simulink model "GFMUPS100k_CPP"  (R2024b)
settings: Solver=ode2  StartTime=0.0  StopTime=6  FixedStep=5e-7  RelTol=1e-3
model workspace (MAT data in the model file):
  amp = 0
  f1 = 1000
undefined symbols (not defined in the file or in its folder): DiscIntNeverNeededParam, L
libraries: spsIGBTDiodeLib x12, slpidlib x12, spsabctodq0Lib x10, spsSeriesRLCBranchLib x9, spsPLL3phLib x8, spsThreePhaseSeriesRLCBranchLib x8, spsDiodeLib x6, dspstat3 x5, spsVoltageMeasurementLib x4, spsThreePhaseVIMeasurementLib x4, spsPower3phInstantaneousLib x3, spsControlledCurrentSourceLib x3
(part 4 of 4)

== matlab function GFMUPS100k_CPP/A practical and fast sequence components detection scheme for three-phase unbalanced grid voltage.2021/Ubeta计算/MATLAB Function9 ==
  data: u_alpha input; u_beta output; Ts input; omega input; N input
function u_beta = MultiPoint_OSG(u_alpha, Ts, omega, N)
% MULTIPOINT_OSG: 基于多点最小二乘最优拟合的正交信号构造
% 
% 参数说明:
%   u_alpha : 当前时刻的单相采样输入 u(k)
%   Ts      : 采样周期 (例如 1e-4)
%   omega   : 电网基波角频率 (例如 2*pi*50)
%   N       : 拟合使用的总点数 (建议值：4 代表4点拟合；21 代表2毫秒全密集拟合)

% 声明持久变量：历史缓冲区、常数系数数组、初始化标志
persistent u_buffer C_coeffs initialized;

% 初始化模块 (仅在系统启动的第一个采样周期执行一次，极大节省算力)
if isempty(initialized)
    % 1. 计算相邻采样点的电角度步长
    alpha = omega * Ts;
    
    % 2. 预生成约束矩阵的三角函数项
    c = zeros(N, 1);
    s = zeros(N, 1);
    for i = 1:N
        c(i) = cos((i-1) * alpha);
        s(i) = sin((i-1) * alpha);
    end
    
    % 3. 计算中间常数矩阵
    M11 = sum(c.^2);
    M12 = sum(c .* s);
    M22 = sum(s.^2);
    Delta = M11 * M22 - M12^2;
    
    % 4. 计算最优抗噪系数 C0, C1 ... C_N-1
    C_coeffs = zeros(N, 1);
    for i = 1:N
        C_coeffs(i) = (M12 * c(i) - M11 * s(i)) / Delta;
    end
    
    % 【极性匹配说明】
    % 您原先的代码 u_beta = (u(k-1) - u(k)*cos)/sin 
    % 在输入为 sin(wt) 时，输出的是 -cos(wt)。
    % 为了确保替换后系统后续的 PLL 或控制逻辑不受极性翻转的影响，这里乘以 -1。
    C_coeffs = -C_coeffs; 
    
    % 5. 初始化历史数据移位寄存器 (全 0)
    u_buffer = zeros(N, 1);
    initialized = true;
end

% ================= 实 时 运 行 区 =================

% 1. 更新历史数据缓冲区 (FIFO 移位)
% 将旧数据向后平移，新数据 u_alpha 推入头部 (u_buffer(1) 代表当前 k 时刻)
for i = N:-1:2
    u_buffer(i) = u_buffer(i-1);
end
u_buffer(1) = u_alpha;

% 2. 核心正交计算 (向量内积乘加运算)
% 等效于: u_beta = C0*u(k) + C1*u(k-1) + C2*u(k-2) + ...
u_beta = sum(C_coeffs .* u_buffer);

end

== matlab function GFMUPS100k_CPP/A practical and fast sequence components detection scheme for three-phase unbalanced grid voltage.2021/Subsystem/MATLAB Function1 ==
  settings: updateMethod=DISCRETE
  data: u input; y_out output
function y_out = maf_filter(u)
    % 滑动平均滤波法 (MAF)
    % 采样时间: 1e-4 s, 电网基波频率: 50 Hz
    % 窗口长度 L: T/2 = 0.01 s -> 100 个采样点 (用于消除 3, 5, 7 次等奇次谐波)
    
    % 定义持久化变量
    persistent buf_maf sum_maf idx_maf
    
    if isempty(buf_maf)
        buf_maf = zeros(100, 1);
        sum_maf = 0;
        idx_maf = 1;
    end
    
    % 读取窗口中最旧的值，即公式 (41) 中的 u(t - L*DeltaT)
    u_old = buf_maf(idx_maf);
    
    % 采用递推方式更新滑动窗口的总和，大幅降低每步运算量
    sum_maf = sum_maf + u - u_old; 
    
    % 计算当前步的平均值
    y_out = sum_maf / 100;
    
    % 更新环形缓冲区
    buf_maf(idx_maf) = u;
    
    % 更新索引
    idx_maf = idx_maf + 1;
    if idx_maf > 100
        idx_maf = 1;
    end
end

== matlab function GFMUPS100k_CPP/A practical and fast sequence components detection scheme for three-phase unbalanced grid voltage.2021/Subsystem/MATLAB Function2 ==
  settings: updateMethod=DISCRETE
  data: u input; y_out output
function y_out = maf_filter(u)
    % 滑动平均滤波法 (MAF)
    % 采样时间: 1e-4 s, 电网基波频率: 50 Hz
    % 窗口长度 L: T/2 = 0.01 s -> 100 个采样点 (用于消除 3, 5, 7 次等奇次谐波)
    
    % 定义持久化变量
    persistent buf_maf sum_maf idx_maf
    
    if isempty(buf_maf)
        buf_maf = zeros(100, 1);
        sum_maf = 0;
        idx_maf = 1;
    end
    
    % 读取窗口中最旧的值，即公式 (41) 中的 u(t - L*DeltaT)
    u_old = buf_maf(idx_maf);
    
    % 采用递推方式更新滑动窗口的总和，大幅降低每步运算量
    sum_maf = sum_maf + u - u_old; 
    
    % 计算当前步的平均值
    y_out = sum_maf / 100;
    
    % 更新环形缓冲区
    buf_maf(idx_maf) = u;
    
    % 更新索引
    idx_maf = idx_maf + 1;
    if idx_maf > 100
        idx_maf = 1;
    end
end

== matlab function GFMUPS100k_CPP/A practical and fast sequence components detection scheme for three-phase unbalanced grid voltage.2021/MATLAB Function1 ==
  data: Ud_pos input; Mag_pos output; Uq_pos input; Angle_pos output; Mag_neg output; Angle_neg output; Ud_neg input; Uq_neg input; wt input
function [Mag_pos, Angle_pos, Mag_neg, Angle_neg] = Component_Calc_DQ(Ud_pos, Uq_pos, Ud_neg, Uq_neg, wt)
% 输入: 
%   Ud_pos, Uq_pos: 经过滤波后的正序电压 dq 轴分量
%   Ud_neg, Uq_neg: 经过滤波后的负序电压 dq 轴分量
%   wt: 当前的电网同步相位 (omega * t, 弧度)。
% 输出:
%   Mag_pos:   正序幅值
%   Angle_pos: 正序同步相角 (弧度 rad, 范围 0 ~ 2*pi，对应论文的 v+)
%   Mag_neg:   负序幅值
%   Angle_neg: 负序同步相角 (弧度 rad, 范围 0 ~ 2*pi，对应论文的 v-)

% ==========================
% 1. 正序分量计算 (Positive Sequence)
% ==========================
% 根据论文公式(38)计算幅值
Mag_pos = sqrt(Ud_pos^2 + Uq_pos^2);
% 使用 atan2 直接求出初始相角 lambda (对应论文公式31，范围 -pi ~ pi)
lambda = atan2(Uq_pos, Ud_pos);
% 根据论文公式(36)和(37)，计算带有 wt 的实时同步相位 v+
Angle_pos = mod(wt + lambda, 2*pi);

% ==========================
% 2. 负序分量计算 (Negative Sequence)
% ==========================
% 根据论文公式(38)计算幅值
Mag_neg = sqrt(Ud_neg^2 + Uq_neg^2);

% 【新增逻辑】：设定负序幅值死区阈值 (Deadband Threshold)
% 这里的 0.01 代表 1% 的额定电压，你可以根据实际电网的噪声水平微调 (通常在 0.005 ~ 0.02 之间)
epsilon = 0.01; 

if Mag_neg < epsilon
    % 当负序幅值极小时（如电网平衡状态），认为负序不存在，将其相角强制锁定为 0
    Angle_neg = 0;
else
    % 当发生不对称故障，负序幅值越过阈值时，正常计算实时相角
    delta = atan2(Uq_neg, Ud_neg);
    Angle_neg = mod(wt + delta, 2*pi);
end

end

== matlab function GFMUPS100k_CPP/A practical and fast sequence components detection scheme for three-phase unbalanced grid voltage.2021/Subsystem1/MATLAB Function2 ==
  settings: updateMethod=DISCRETE
  data: u input; y_out output
function y_out = maf_filter(u)
    % 滑动平均滤波法 (MAF)
    % 采样时间: 1e-4 s, 电网基波频率: 50 Hz
    % 窗口长度 L: T/2 = 0.01 s -> 100 个采样点 (用于消除 3, 5, 7 次等奇次谐波)
    
    % 定义持久化变量
    persistent buf_maf sum_maf idx_maf
    
    if isempty(buf_maf)
        buf_maf = zeros(100, 1);
        sum_maf = 0;
        idx_maf = 1;
    end
    
    % 读取窗口中最旧的值，即公式 (41) 中的 u(t - L*DeltaT)
    u_old = buf_maf(idx_maf);
    
    % 采用递推方式更新滑动窗口的总和，大幅降低每步运算量
    sum_maf = sum_maf + u - u_old; 
    
    % 计算当前步的平均值
    y_out = sum_maf / 100;
    
    % 更新环形缓冲区
    buf_maf(idx_maf) = u;
    
    % 更新索引
    idx_maf = idx_maf + 1;
    if idx_maf > 100
        idx_maf = 1;
    end
end

== matlab function GFMUPS100k_CPP/SVPWM调制/SVPWM/参考矢量 ==
  data: ua input; Uref output; ub input; uc input
function Uref = V(ua,ub,uc)
Uref=(2/3)*(ua+ub*exp(1i*pi*2/3)+uc*exp(-1i*pi*2/3));

== matlab function GFMUPS100k_CPP/SVPWM调制/SVPWM/小扇区 ==
  data: m input; n output; theta input
function n = SmallVector(m,theta)
LBD=-0.5+m*sin(theta);
LAB=sqrt(3)*m*cos(theta)+m*sin(theta)-1;
LAD=-sqrt(3)*m*cos(theta)+m*sin(theta)+1;
if(theta<pi/6)
    if(LAB<=0)
        n=1;
    elseif(LAD<=0)
        n=5;
    else
        n=3;
    end
else
    if(LAB<=0)
        n=2;
    elseif(LBD>=0)
        n=6;
    else
        n=4;
    end
end

== matlab function GFMUPS100k_CPP/SVPWM调制/SVPWM/矢量作用时间 ==
  data: n input; m input; Ts input; TA output; theta input; TB output; TC output
function [TA,TB,TC] = Vectortime(n,m,Ts,theta)
TA=0;
TB=0;
TC=0;
if(n==1||n==2)
    TA=2*m*Ts*sin(theta);
    TB=Ts*(1-2*m*sin(pi/3+theta));
    TC=2*m*Ts*sin(pi/3-theta);
end
if(n==3||n==4)
    TA=Ts*(1-2*m*sin(theta));
    TB=Ts*(2*m*sin(pi/3+theta)-1);
    TC=Ts*(1-2*m*sin(pi/3-theta));
end
if(n==5)
    TA=2*m*Ts*sin(theta);
    TB=2*Ts*(1-m*sin(pi/3+theta));
    TC=Ts*(2*m*sin(pi/3-theta)-1);
end
if(n==6)
    TA=Ts*(2*m*sin(theta)-1);
    TB=2*Ts*(1-m*sin(pi/3+theta));
    TC=Ts*2*m*sin(pi/3-theta);
end

== matlab function GFMUPS100k_CPP/SVPWM调制/SVPWM/上半周期时间逻辑 ==
  data: TA input; TB input; TC input; n input; t1 output; t2 output; t3 output
function [t1,t2,t3] = timeshare(TA,TB,TC,n)
t1=0;
t2=0;
t3=0;
if(n==1)
    t1=TC;
    t2=TA;
    t3=TB;
end
if(n==2)
    t1=TA;
    t2=TB;
    t3=TC;
end
if(n==3)
    t1=TA;
    t2=TC;
    t3=TB;
end
if(n==4)
    t1=TC;
    t2=TB;
    t3=TA;
end
if(n==5)
    t1=TB;
    t2=TC;
    t3=TA;
end
if(n==6)
    t1=TB;
    t2=TC;
    t3=TA;
end

== matlab function GFMUPS100k_CPP/SVPWM调制/SVPWM/下半周期时间逻辑 ==
  data: TA input; TB input; TC input; n input; t1 output; t2 output; t3 output
function [t1,t2,t3] = timeshare(TA,TB,TC,n)
t1=0;
t2=0;
t3=0;
if(n==1)
    t1=TC;
    t2=TB;
    t3=TA;
end
if(n==2)
    t1=TA;
    t2=TC;
    t3=TB;
end
if(n==3)
    t1=TA;
    t2=TB;
    t3=TC;
end
if(n==4)
    t1=TC;
    t2=TA;
    t3=TB;
end
if(n==5)
    t1=TB;
    t2=TA;
    t3=TC;
end
if(n==6)
    t1=TB;
    t2=TA;
    t3=TC;
end

== matlab function GFMUPS100k_CPP/SVPWM调制/SVPWM/按规律选择 ==
  data: ta1 input; tb1 input; tc1 input; ta2 input; T1 output; T2 output; T3 output; tb2 input; tc2 input; N input
function [T1,T2,T3] = switchshare(ta1,tb1,tc1,ta2,tb2,tc2,N)
T1=0;
T2=0;
T3=0;
if(N==1)
    T1=ta1;
    T2=tb1;
    T3=tc1;
end
if(N==2)
    T1=ta2;
    T2=tb2;
    T3=tc2;
end
if(N==3)
    T1=ta1;
    T2=tb1;
    T3=tc1;
end
if(N==4)
    T1=ta2;
    T2=tb2;
    T3=tc2;
end
if(N==5)
    T1=ta1;
    T2=tb1;
    T3=tc1;
end
if(N==6)
    T1=ta2;
    T2=tb2;
    T3=tc2;
end
